simulink model "solar_pv_protected_c07_circuit"  (R2026b)
settings: Solver=VariableStepAuto
model workspace (MAT data in the model file):
  candidate_owner = 'pv_protection_integration_20261023_r01'
  solar_edit_metadata : object (value not decoded)
libraries: fl_lib x149, ee_lib x16, ltc4364demo_lib x3, batteryecm_lib x1, solarprotect_lib x1
(part 10 of 16)

== system solar_pv_protected_c07_circuit/PV1 ==
  Pin_001 : PMIOPort  Description=|  Side=Left  ConnectionType=Connection: foundation.electrical.electrical
      | 識別名　　　　　　　; Pin_001
      | 種別　　　　　　　　; Simscape Connection Port（階層境界の物理端子）
      | 所属部品　　　　　　; PV1
      | 配置目的　　　　　　; 内部の電気ノードを、この外箱の外側の対応端子へ引き出す。
      | 対応端子　　　　　　; lconn:1／-番 -
      | 接続ラベル　　　　　; GND、PROT_RETURN
      | モデルの範囲　　　　; 実部品を1個追加する表現ではない。端子自体に増幅・遮断・測定機能を持たない。
      | 端子番号の注意　　　; Connection Portの番号は外箱内の対応番号であり、実パッケージのピン番号とは区別する。
      | 確認の範囲　　　　　; 実ポートと階層対応による静的接続の説明。電気特性の再現性は所属部品の説明を参照する。
      | 
      | 従来の補足　　　　　; 以前のDescriptionを以下に保持する。
      | Physical PV1 pin - / -
      | 
      | 【この説明欄の略語・記号】
      | 用語1　　　　　　　 ; GND：Ground（回路の基準電位・電流帰路）。この図の共通基準。保護接地や大地への接続を意味するとは限らない。
      | 用語2　　　　　　　 ; PROT_RETURN：保護回路の共通帰路。PROTはProtection（保護）、RETURNは帰路。プロトタイプの略ではなく、現回路では共通GNDへつながる。
  Pin_002 : PMIOPort  Description=|  Port=2  Side=Right  ConnectionType=Connection: foundation.electrical.electrical
      | 識別名　　　　　　　; Pin_002
      | 種別　　　　　　　　; Simscape Connection Port（階層境界の物理端子）
      | 所属部品　　　　　　; PV1
      | 配置目的　　　　　　; 内部の電気ノードを、この外箱の外側の対応端子へ引き出す。
      | 対応端子　　　　　　; rconn:1／+番 +
      | 接続ラベル　　　　　; ラベルなし。接続は実線と境界対応で定義する。
      | モデルの範囲　　　　; 実部品を1個追加する表現ではない。端子自体に増幅・遮断・測定機能を持たない。
      | 端子番号の注意　　　; Connection Portの番号は外箱内の対応番号であり、実パッケージのピン番号とは区別する。
      | 確認の範囲　　　　　; 実ポートと階層対応による静的接続の説明。電気特性の再現性は所属部品の説明を参照する。
      | 
      | 従来の補足　　　　　; 以前のDescriptionを以下に保持する。
      | Physical PV1 pin + / +

== system solar_pv_protected_c07_circuit/PV2 ==
  Pin_001 : PMIOPort  Description=|  Side=Left  ConnectionType=Connection: foundation.electrical.electrical
      | 識別名　　　　　　　; Pin_001
      | 種別　　　　　　　　; Simscape Connection Port（階層境界の物理端子）
      | 所属部品　　　　　　; PV2
      | 配置目的　　　　　　; 内部の電気ノードを、この外箱の外側の対応端子へ引き出す。
      | 対応端子　　　　　　; lconn:1／-番 -
      | 接続ラベル　　　　　; ラベルなし。接続は実線と境界対応で定義する。
      | モデルの範囲　　　　; 実部品を1個追加する表現ではない。端子自体に増幅・遮断・測定機能を持たない。
      | 端子番号の注意　　　; Connection Portの番号は外箱内の対応番号であり、実パッケージのピン番号とは区別する。
      | 確認の範囲　　　　　; 実ポートと階層対応による静的接続の説明。電気特性の再現性は所属部品の説明を参照する。
      | 
      | 従来の補足　　　　　; 以前のDescriptionを以下に保持する。
      | Physical PV2 pin - / -
  Pin_002 : PMIOPort  Description=|  Port=2  Side=Right  ConnectionType=Connection: foundation.electrical.electrical
      | 識別名　　　　　　　; Pin_002
      | 種別　　　　　　　　; Simscape Connection Port（階層境界の物理端子）
      | 所属部品　　　　　　; PV2
      | 配置目的　　　　　　; 内部の電気ノードを、この外箱の外側の対応端子へ引き出す。
      | 対応端子　　　　　　; rconn:1／+番 +
      | 接続ラベル　　　　　; ラベルなし。接続は実線と境界対応で定義する。
      | モデルの範囲　　　　; 実部品を1個追加する表現ではない。端子自体に増幅・遮断・測定機能を持たない。
      | 端子番号の注意　　　; Connection Portの番号は外箱内の対応番号であり、実パッケージのピン番号とは区別する。
      | 確認の範囲　　　　　; 実ポートと階層対応による静的接続の説明。電気特性の再現性は所属部品の説明を参照する。
      | 
      | 従来の補足　　　　　; 以前のDescriptionを以下に保持する。
      | Physical PV2 pin + / +
